simulink model "Reformable_AI_2025"  (R2025b)
settings: Solver=ode23t  StartTime=0.0  StopTime=150  FixedStep=0.01  RelTol=1e-3
InitFcn:
  | load('PV_Params_Stage1.mat'); load('PV_Params_Stage2.mat');
values from neighbouring files (symbols this model uses):
  Iph_ref = P.Iph_ref*(1 - K.k_Iph*D)    [PaperFigures.m]
  n = lower(name)    [Stage10C_inventory.m]    (also in Stage10F2_make_manifest.m = size(rows,1); Stage10F_make_manifest.m = size(rows,1); Stage10F_run_one.m = 1; Stage10_assemble_dataset.m = height(T))
  OCV_tbl = [11.6 11.8 11.9 12.1 12.2 12.3 12.4 12.5 12.6 12.7 12.8]    [Battery_Param_Definition.m]
  Q = 7    [Battery_Param_Definition.m]
  q = 1.602176634e-19    [PaperFigures.m]    (also in Stage10C_inventory.m = L(strcmp({L.folder}, fl{k})); Stage10F2_make_manifest.m = M(M.regime == "A" & abs(M.bD - L) < 1e-12, :); Stage10F_make_manifest.m = M(M.regime == "A" & abs(M.bD - L) < 1e-12, :); Stage10G2_final_test.m = zeros(1, numel(seeds)))
  R0 = 0.03    [Battery_Param_Definition.m]    (also in PaperFigures.m = B.R0*(1 + KB.k_R0*D))
  R1 = 0.015    [Battery_Param_Definition.m]    (also in PaperFigures.m = B.R1*(1 + KB.k_R1*D))
  Rs = P.Rs*(1 + K.k_Rs*D)    [PaperFigures.m]
  Rsh = P.Rsh*(1 - K.k_Rsh*D)    [PaperFigures.m]
  SOC_bp = [0 10 20 30 40 50 60 70 80 90 100]    [Battery_Param_Definition.m]
  SOC_init = 100    [Battery_Param_Definition.m]
undefined symbols (not defined in the file or in its folder): Battery_Twin_C1, Battery_Twin_Capacity, Battery_Twin_OCV_tbl, Battery_Twin_R0, Battery_Twin_R1, Battery_Twin_SOC_bp, Battery_Twin_SOC_init, Battery_Twin_Vp_init, bias_G, bias_I_batt, bias_I_pv, bias_T_batt, bias_Tc, bias_V_batt, bias_V_pv, dG, dI_batt, dI_pv, drift_G, drift_I_batt, drift_I_pv, drift_T_batt, drift_Tc, drift_V_batt, drift_V_pv, dT_batt, dTc, dV_batt, dV_pv, Eg, ExcessiveNoise_Sigma, ExcessiveNoise_Sigma_batt, ExtraDrift_Rate, ExtraDrift_Rate_batt, FaultBias_Value, FaultBias_Value_batt, FaultSat_Max, FaultSat_Max_batt, FaultSat_Min, FaultSat_Min_batt, G_max, G_min, Gref, I0_ref, I_batt_max, I_batt_min, I_pv_max, I_pv_min, IntermittentDropoutProb, IntermittentDropoutProb_batt, Isc_ref, k_B, k_Iph, k_Q, k_R0, k_R1, k_Rs, k_Rsh, Ki, noise_G ... (+44)
libraries: fl_lib x7, nesl_utility x6
(part 2 of 3)

== system Reformable_AI_2025/PV_Resdual_Model ==
  PV_Twin_Current : Inport
  PV_Twin_Power : Inport  Port=2
  PV_Measured_Power : Inport  Port=3
  PV_Measured_Current : Inport  Port=4
  MATLAB Function : MATLAB Function  TreatAsAtomicUnit=on
  To Workspace : ToWorkspace  VariableName=PV_Residual_Current  SaveFormat=Timeseries  SampleTime=-1
  To Workspace1 : ToWorkspace  VariableName=PV_Residual_Power  SaveFormat=Timeseries  SampleTime=-1
  PV_Residual_Current : Outport
  PV_Residual_Power : Outport  Port=2
  wires:
  PV_Twin_Power/1 -> MATLAB Function/4(PV_Twin_Power)
  PV_Measured_Power/1 -> MATLAB Function/3(PV_Measured_Power)
  PV_Twin_Current/1 -> MATLAB Function/2(PV_Twin_Current)
  PV_Measured_Current/1 -> MATLAB Function/1(PV_Measured_Current)
  MATLAB Function/1(PV_Residual_Current) -> To Workspace/1, PV_Residual_Current/1
  MATLAB Function/2(PV_Residual_Power) -> To Workspace1/1, PV_Residual_Power/1

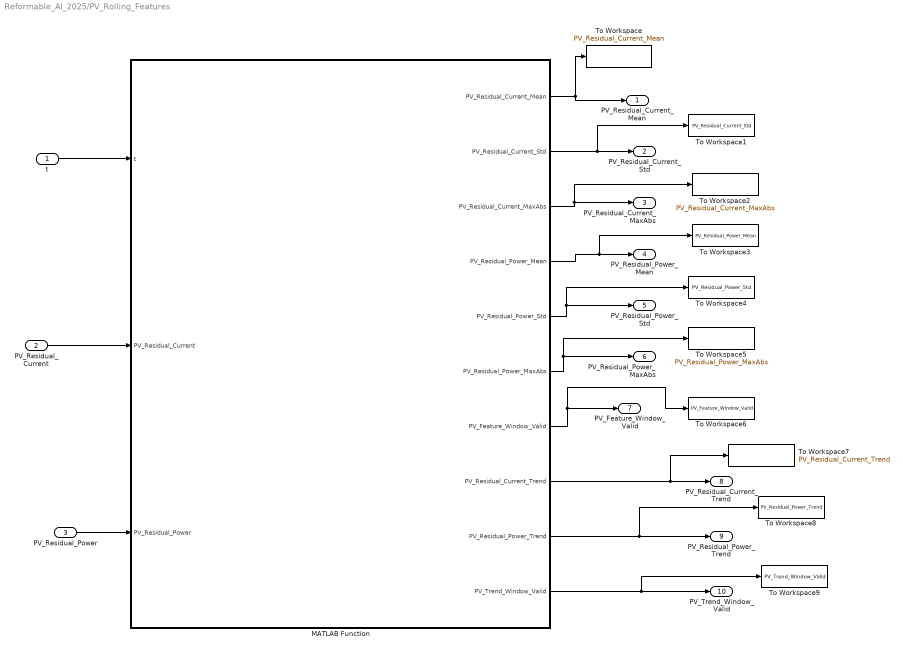
== system Reformable_AI_2025/PV_Rolling_Features ==
  t : Inport
  PV_Residual_Current : Inport  Port=2
  PV_Residual_Power : Inport  Port=3
  MATLAB Function : MATLAB Function  TreatAsAtomicUnit=on  SystemSampleTime=Stage9_Feature_SampleTime
  To Workspace : ToWorkspace  VariableName=PV_Residual_Current_Mean  SaveFormat=Timeseries  SampleTime=-1
  To Workspace1 : ToWorkspace  VariableName=PV_Residual_Current_Std  SaveFormat=Timeseries  SampleTime=-1
  To Workspace2 : ToWorkspace  VariableName=PV_Residual_Current_MaxAbs  SaveFormat=Timeseries  SampleTime=-1
  To Workspace3 : ToWorkspace  VariableName=PV_Residual_Power_Mean  SaveFormat=Timeseries  SampleTime=-1
  To Workspace4 : ToWorkspace  VariableName=PV_Residual_Power_Std  SaveFormat=Timeseries  SampleTime=-1
  To Workspace5 : ToWorkspace  VariableName=PV_Residual_Power_MaxAbs  SaveFormat=Timeseries  SampleTime=-1
  To Workspace6 : ToWorkspace  VariableName=PV_Feature_Window_Valid  SaveFormat=Timeseries  SampleTime=-1
  To Workspace7 : ToWorkspace  VariableName=PV_Residual_Current_Trend  SaveFormat=Timeseries  SampleTime=-1
  To Workspace8 : ToWorkspace  VariableName=PV_Residual_Power_Trend  SaveFormat=Timeseries  SampleTime=-1
  To Workspace9 : ToWorkspace  VariableName=PV_Trend_Window_Valid  SaveFormat=Timeseries  SampleTime=-1
  PV_Residual_Current_Mean : Outport
  PV_Residual_Current_Std : Outport  Port=2
  PV_Residual_Current_MaxAbs : Outport  Port=3
  PV_Residual_Power_Mean : Outport  Port=4
  PV_Residual_Power_Std : Outport  Port=5
  PV_Residual_Power_MaxAbs : Outport  Port=6
  PV_Feature_Window_Valid : Outport  Port=7
  PV_Residual_Current_Trend : Outport  Port=8
  PV_Residual_Power_Trend : Outport  Port=9
  PV_Trend_Window_Valid : Outport  Port=10
  wires:
  t/1 -> MATLAB Function/1(t)
  PV_Residual_Current/1 -> MATLAB Function/2(PV_Residual_Current)
  PV_Residual_Power/1 -> MATLAB Function/3(PV_Residual_Power)
  MATLAB Function/1(PV_Residual_Current_Mean) -> To Workspace/1, PV_Residual_Current_Mean/1
  MATLAB Function/2(PV_Residual_Current_Std) -> To Workspace1/1, PV_Residual_Current_Std/1
  MATLAB Function/3(PV_Residual_Current_MaxAbs) -> To Workspace2/1, PV_Residual_Current_MaxAbs/1
  MATLAB Function/4(PV_Residual_Power_Mean) -> To Workspace3/1, PV_Residual_Power_Mean/1
  MATLAB Function/5(PV_Residual_Power_Std) -> To Workspace4/1, PV_Residual_Power_Std/1
  MATLAB Function/6(PV_Residual_Power_MaxAbs) -> To Workspace5/1, PV_Residual_Power_MaxAbs/1
  MATLAB Function/7(PV_Feature_Window_Valid) -> To Workspace6/1, PV_Feature_Window_Valid/1
  MATLAB Function/8(PV_Residual_Current_Trend) -> To Workspace7/1, PV_Residual_Current_Trend/1
  MATLAB Function/9(PV_Residual_Power_Trend) -> To Workspace8/1, PV_Residual_Power_Trend/1
  MATLAB Function/10(PV_Trend_Window_Valid) -> To Workspace9/1, PV_Trend_Window_Valid/1

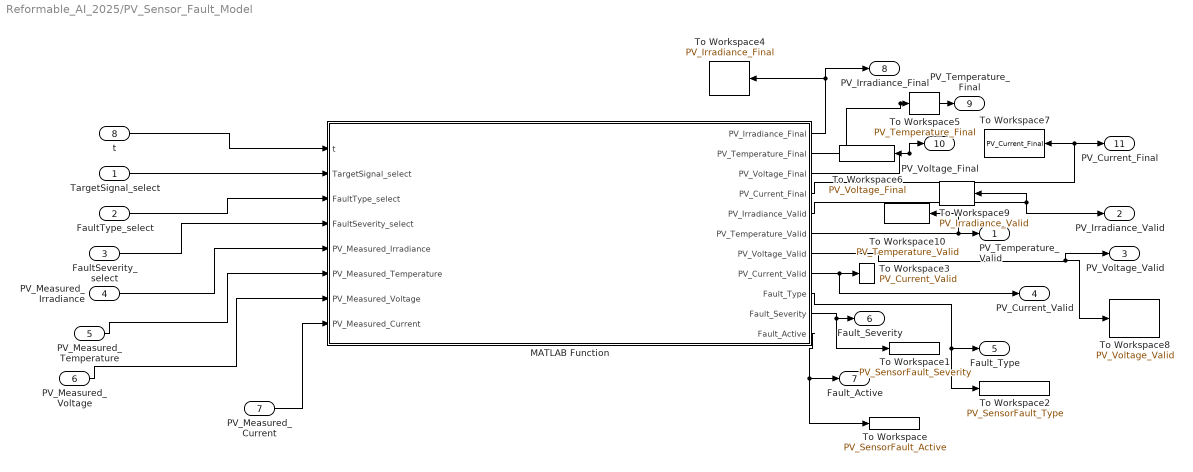
== system Reformable_AI_2025/PV_Sensor_Fault_Model ==
  TargetSignal_select : Inport
  FaultType_select : Inport  Port=2
  FaultSeverity_select : Inport  Port=3
  PV_Measured_Irradiance : Inport  Port=4
  PV_Measured_Temperature : Inport  Port=5
  PV_Measured_Voltage : Inport  Port=6
  PV_Measured_Current : Inport  Port=7
  t : Inport  Port=8
  MATLAB Function : MATLAB Function  TreatAsAtomicUnit=on
  To Workspace : ToWorkspace  VariableName=PV_SensorFault_Active  SaveFormat=Timeseries  SampleTime=-1
  To Workspace1 : ToWorkspace  VariableName=PV_SensorFault_Severity  SaveFormat=Timeseries  SampleTime=-1
  To Workspace10 : ToWorkspace  VariableName=PV_Temperature_Valid  SaveFormat=Timeseries  SampleTime=-1
  To Workspace2 : ToWorkspace  VariableName=PV_SensorFault_Type  SaveFormat=Timeseries  SampleTime=-1
  To Workspace3 : ToWorkspace  VariableName=PV_Current_Valid  SaveFormat=Timeseries  SampleTime=-1
  To Workspace4 : ToWorkspace  VariableName=PV_Irradiance_Final  SaveFormat=Timeseries  SampleTime=-1
  To Workspace5 : ToWorkspace  VariableName=PV_Temperature_Final  SaveFormat=Timeseries  SampleTime=-1
  To Workspace6 : ToWorkspace  VariableName=PV_Voltage_Final  SaveFormat=Timeseries  SampleTime=-1
  To Workspace7 : ToWorkspace  VariableName=PV_Current_Final  SaveFormat=Timeseries  SampleTime=-1
  To Workspace8 : ToWorkspace  VariableName=PV_Voltage_Valid  SaveFormat=Timeseries  SampleTime=-1
  To Workspace9 : ToWorkspace  VariableName=PV_Irradiance_Valid  SaveFormat=Timeseries  SampleTime=-1
  PV_Temperature_Valid : Outport
  PV_Irradiance_Valid : Outport  Port=2
  PV_Voltage_Valid : Outport  Port=3
  PV_Current_Valid : Outport  Port=4
  Fault_Type : Outport  Port=5
  Fault_Severity : Outport  Port=6
  Fault_Active : Outport  Port=7
  PV_Irradiance_Final : Outport  Port=8
  PV_Temperature_Final : Outport  Port=9
  PV_Voltage_Final : Outport  Port=10
  PV_Current_Final : Outport  Port=11
  wires:
  t/1 -> MATLAB Function/1(t)
  TargetSignal_select/1 -> MATLAB Function/2(TargetSignal_select)
  FaultType_select/1 -> MATLAB Function/3(FaultType_select)
  FaultSeverity_select/1 -> MATLAB Function/4(FaultSeverity_select)
  PV_Measured_Irradiance/1 -> MATLAB Function/5(PV_Measured_Irradiance)
  PV_Measured_Temperature/1 -> MATLAB Function/6(PV_Measured_Temperature)
  PV_Measured_Voltage/1 -> MATLAB Function/7(PV_Measured_Voltage)
  PV_Measured_Current/1 -> MATLAB Function/8(PV_Measured_Current)
  MATLAB Function/1(PV_Irradiance_Final) -> To Workspace4/1, PV_Irradiance_Final/1
  MATLAB Function/2(PV_Temperature_Final) -> To Workspace5/1, PV_Temperature_Final/1
  MATLAB Function/3(PV_Voltage_Final) -> PV_Voltage_Final/1, To Workspace6/1
  MATLAB Function/4(PV_Current_Final) -> PV_Current_Final/1, To Workspace7/1
  MATLAB Function/5(PV_Irradiance_Valid) -> PV_Irradiance_Valid/1, To Workspace9/1
  MATLAB Function/6(PV_Temperature_Valid) -> To Workspace10/1, PV_Temperature_Valid/1
  MATLAB Function/7(PV_Voltage_Valid) -> To Workspace8/1, PV_Voltage_Valid/1
  MATLAB Function/8(PV_Current_Valid) -> PV_Current_Valid/1, To Workspace3/1
  MATLAB Function/9(Fault_Type) -> Fault_Type/1, To Workspace2/1
  MATLAB Function/10(Fault_Severity) -> To Workspace1/1, Fault_Severity/1
  MATLAB Function/11(Fault_Active) -> Fault_Active/1, To Workspace/1

== system Reformable_AI_2025/PV_Twin_Valid_Operating_Point ==
  PV_Measured_Voltage : Inport
  PV_Measured_Irradiance : Inport  Port=2
  PV_Twin_Current : Inport  Port=3
  PV_Twin_Power : Inport  Port=4
  MATLAB Function : MATLAB Function  TreatAsAtomicUnit=on
  To Workspace : ToWorkspace  VariableName=PV_Twin_Valid_Operating_Point  SaveFormat=Timeseries  SampleTime=-1
  PV_Twin_Valid_Operating_Point : Outport
  wires:
  MATLAB Function/1(PV_Twin_Valid_Operating_Point) -> To Workspace/1, PV_Twin_Valid_Operating_Point/1
  PV_Measured_Voltage/1 -> MATLAB Function/1(PV_Measured_Voltage)
  PV_Measured_Irradiance/1 -> MATLAB Function/2(PV_Measured_Irradiance)
  PV_Twin_Current/1 -> MATLAB Function/3(PV_Twin_Current)
  PV_Twin_Power/1 -> MATLAB Function/4(PV_Twin_Power)

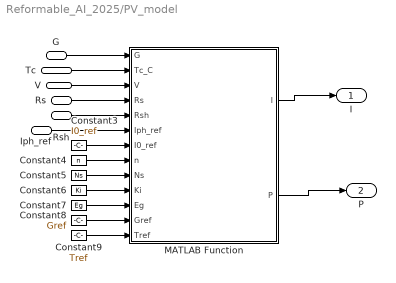
== system Reformable_AI_2025/PV_model ==
  G : Inport
  Tc : Inport  Port=2
  V : Inport  Port=3
  Rs : Inport  Port=4
  Rsh : Inport  Port=5
  Iph_ref : Inport  Port=6
  Constant3 : Constant  Value=I0_ref
  Constant4 : Constant  Value=n
  Constant5 : Constant  Value=Ns
  Constant6 : Constant  Value=Ki
  Constant7 : Constant  Value=Eg
  Constant8 : Constant  Value=Gref
  Constant9 : Constant  Value=Tref
  MATLAB Function : MATLAB Function  TreatAsAtomicUnit=on
  I : Outport
  P : Outport  Port=2
  wires:
  MATLAB Function/1(I) -> I/1
  G/1 -> MATLAB Function/1(G)
  Tc/1 -> MATLAB Function/2(Tc_C)
  V/1 -> MATLAB Function/3(V)
  MATLAB Function/2(P) -> P/1
  Rs/1 -> MATLAB Function/4(Rs)
  Rsh/1 -> MATLAB Function/5(Rsh)
  Iph_ref/1 -> MATLAB Function/6(Iph_ref)
  Constant3/1 -> MATLAB Function/7(I0_ref)
  Constant4/1 -> MATLAB Function/8(n)
  Constant5/1 -> MATLAB Function/9(Ns)
  Constant6/1 -> MATLAB Function/10(Ki)
  Constant7/1 -> MATLAB Function/11(Eg)
  Constant9/1 -> MATLAB Function/13(Tref)
  Constant8/1 -> MATLAB Function/12(Gref)

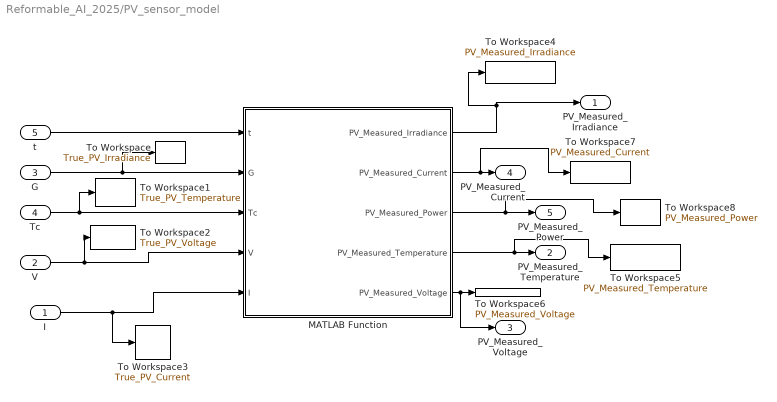
== system Reformable_AI_2025/PV_sensor_model ==
  I : Inport
  V : Inport  Port=2
  G : Inport  Port=3
  Tc : Inport  Port=4
  t : Inport  Port=5
  MATLAB Function : MATLAB Function  TreatAsAtomicUnit=on
  To Workspace : ToWorkspace  VariableName=True_PV_Irradiance  SaveFormat=Timeseries  SampleTime=-1
  To Workspace1 : ToWorkspace  VariableName=True_PV_Temperature  SaveFormat=Timeseries  SampleTime=-1
  To Workspace2 : ToWorkspace  VariableName=True_PV_Voltage  SaveFormat=Timeseries  SampleTime=-1
  To Workspace3 : ToWorkspace  VariableName=True_PV_Current  SaveFormat=Timeseries  SampleTime=-1
  To Workspace4 : ToWorkspace  VariableName=PV_Measured_Irradiance  SaveFormat=Timeseries  SampleTime=-1
  To Workspace5 : ToWorkspace  VariableName=PV_Measured_Temperature  SaveFormat=Timeseries  SampleTime=-1
  To Workspace6 : ToWorkspace  VariableName=PV_Measured_Voltage  SaveFormat=Timeseries  SampleTime=-1
  To Workspace7 : ToWorkspace  VariableName=PV_Measured_Current  SaveFormat=Timeseries  SampleTime=-1
  To Workspace8 : ToWorkspace  VariableName=PV_Measured_Power  SaveFormat=Timeseries  SampleTime=-1
  PV_Measured_Irradiance : Outport
  PV_Measured_Temperature : Outport  Port=2
  PV_Measured_Voltage : Outport  Port=3
  PV_Measured_Current : Outport  Port=4
  PV_Measured_Power : Outport  Port=5
  wires:
  Tc/1 -> To Workspace1/1, MATLAB Function/3(Tc)
  G/1 -> To Workspace/1, MATLAB Function/2(G)
  V/1 -> To Workspace2/1, MATLAB Function/4(V)
  t/1 -> MATLAB Function/1(t)
  MATLAB Function/1(PV_Measured_Irradiance) -> To Workspace4/1, PV_Measured_Irradiance/1
  I/1 -> To Workspace3/1, MATLAB Function/5(I)
  MATLAB Function/5(PV_Measured_Voltage) -> PV_Measured_Voltage/1, To Workspace6/1
  MATLAB Function/2(PV_Measured_Current) -> To Workspace7/1, PV_Measured_Current/1
  MATLAB Function/3(PV_Measured_Power) -> To Workspace8/1, PV_Measured_Power/1
  MATLAB Function/4(PV_Measured_Temperature) -> To Workspace5/1, PV_Measured_Temperature/1

== matlab function Reformable_AI_2025/PV_Fault_Model/MATLAB Function ==
  data: t input; Rs_fault output; Rs_aged input; Rsh_aged input; Iph_ref_aged input; FaultType_select input; FaultSeverity_select input; Rsh_fault output; Iph_fault output; Fault_Type output; Fault_Severity output; Fault_Active output; Fault_TempRise output
function [Rs_fault, Rsh_fault, Iph_fault, Fault_Type, Fault_Severity, Fault_Active, Fault_TempRise] = ...
    fcn(t, Rs_aged, Rsh_aged, Iph_ref_aged, FaultType_select, FaultSeverity_select)

% TwinAdapt-PHM Stage 5: PV Fault Injection
% Faults modify DEGRADED (aged) parameters, never nameplate/reference values.
% FaultType_select: 0=Healthy 1=Shading 2=Soiling 3=Hotspot 4=PID 5=OpenCircuit 6=ShortCircuit
% FaultSeverity_select: 0 (no fault) to 1 (fully severe)

s = max(0, min(1, FaultSeverity_select));  % clamp severity to [0,1]
ft = round(FaultType_select);

% Defaults: pass-through (Healthy)
Rs_fault  = Rs_aged;
Rsh_fault = Rsh_aged;
Iph_fault = Iph_ref_aged;
Fault_TempRise = 0;
Fault_Active = (ft ~= 0) && (s > 0);

switch ft

    case 0  % Healthy
        Fault_Type = 0;
        Fault_Severity = 0;

    case 1  % Partial Shading -> reduces Iph
        ShadeFactor = s;                      % up to 100% reduction at s=1
        Iph_fault = Iph_ref_aged * (1 - ShadeFactor);
        Fault_Type = 1;
        Fault_Severity = s;

    case 2  % Soiling -> mild Iph reduction + slight temp rise
        Iph_fault = Iph_ref_aged * (1 - 0.3*s);   % gentler than shading
        Fault_TempRise = 5 * s;                   % degC, gradual heating
        Fault_Type = 2;
        Fault_Severity = s;

    case 3  % Hotspot -> increases Rs, raises temperature
        k_hotspot = 4.0;                          % tunable multiplier gain
        Rs_fault = Rs_aged * (1 + k_hotspot*s);
        Fault_TempRise = 40 * s;                   % degC, hotspots run hot
        Fault_Type = 3;
        Fault_Severity = s;

    case 4  % PID -> collapses Rsh (leakage current path)
        k_pid = 0.95;                              % up to 95% Rsh reduction
        Rsh_fault = Rsh_aged * (1 - k_pid*s);
        Fault_Type = 4;
        Fault_Severity = s;

    case 5  % Open Circuit -> current forced to ~0
        Iph_fault = Iph_ref_aged * (1 - s);         % s=1 -> Iph~0 -> I~0, V~Voc
        Rs_fault = Rs_aged * (1 + 50*s);            % huge series resistance emulates open ckt
        Fault_Type = 5;
        Fault_Severity = s;

    case 6  % Short Circuit -> voltage forced to ~0
        Rsh_fault = Rsh_aged * (1 - 0.999*s);       % Rsh -> ~0 collapses voltage
        Fault_Type = 6;
        Fault_Severity = s;

    otherwise  % unrecognized code -> treat as Healthy, flag inactive
        Fault_Type = 0;
        Fault_Severity = 0;
        Fault_Active = false;
end

end

== matlab function Reformable_AI_2025/Battery_Fault_Model/MATLAB Function ==
  data: t input; R0_fault output; R0_aged input; R1_aged input; Q input; OCV_delta input; D_batt input; H_batt input; Battery_Health_State input; FaultType_select input; FaultSeverity_select input; R1_fault output; Q_fault output; OCV_delta_fault output; D_batt output; H_batt output; Battery_Health_State output; Fault_Type output; Fault_Severity output; Fault_Active output; Battery_TempRise output; Safety_Flag output; SafetyFlag_Warning_ThresholdC parameter; SafetyFlag_Critical_ThresholdC parameter; SafetyFlag_Emergency_ThresholdC parameter; k_open_R0 parameter; TempRise_short parameter; k_short_R0 parameter; TempRise_runaway parameter; k_runaway_R0 parameter; TempRise_overcharge parameter; k_overcharge_OCV parameter; k_overcharge_R1 parameter; k_overdischarge_R0 parameter; k_overdischarge_Q parameter; TempRise_overdischarge parameter; TempRise_imbalance parameter; k_imbalance_OCV parameter; k_imbalance_R0 parameter
function [R0_fault, R1_fault, Q_fault, OCV_delta_fault, D_batt, H_batt, ...
          Battery_Health_State, Fault_Type, Fault_Severity, Fault_Active, ...
          Battery_TempRise, Safety_Flag] = ...
    fcn(t, R0_aged, R1_aged, Q, OCV_delta, D_batt, H_batt, ...
          Battery_Health_State, FaultType_select, FaultSeverity_select, ...
        SafetyFlag_Warning_ThresholdC, SafetyFlag_Critical_ThresholdC, SafetyFlag_Emergency_ThresholdC, k_open_R0, ...
TempRise_short, ...
k_short_R0, TempRise_runaway, ...
k_runaway_R0, TempRise_overcharge, ...
k_overcharge_OCV, k_overcharge_R1, k_overdischarge_R0, k_overdischarge_Q, TempRise_overdischarge, ...
TempRise_imbalance, ...
k_imbalance_OCV, k_imbalance_R0)

% TwinAdapt-PHM Stage 6: Battery Fault Injection
% Faults modify DEGRADED (aged) parameters, never nameplate/reference values.
% FaultType_select: 0=Healthy 1=CellImbalance 2=OverDischarge 3=OverCharge
%                   4=ThermalRunawayOnset 5=InternalShort 6=OpenCircuit
%                   7=SensorFault (placeholder -- see note below)
%
% NOTE ON SYMBOLS PANE: everything after FaultSeverity_select in the
% argument list above must have its Scope set to "Parameter" in the
% Ports and Data Manager, NOT "Input". Only the first 10 arguments
% (t through FaultSeverity_select) should be Scope = Input.

s = max(0, min(1, FaultSeverity_select));  % clamp severity to [0,1]
ft = round(FaultType_select);

% Defaults: pass-through (Healthy)
R0_fault         = R0_aged;
R1_fault         = R1_aged;
Q_fault          = Q;
OCV_delta_fault  = OCV_delta;
Battery_TempRise = 0;
Fault_Active     = (ft ~= 0) && (s > 0);

switch ft

    case 0  % Healthy
        Fault_Type = 0;
        Fault_Severity = 0;

    case 1  % Cell Imbalance -> mild R0 rise, OCV uncertainty band
        R0_fault = R0_aged * (1 + k_imbalance_R0*s);
        OCV_delta_fault = OCV_delta + k_imbalance_OCV*s;
        Battery_TempRise = TempRise_imbalance * s;
        Fault_Type = 1;
        Fault_Severity = s;

    case 2  % Over-Discharge -> permanent capacity loss, R0 rise
        Q_fault = Q * (1 - k_overdischarge_Q*s);
        R0_fault = R0_aged * (1 + k_overdischarge_R0*s);
        Battery_TempRise = TempRise_overdischarge * s;
        Fault_Type = 2;
        Fault_Severity = s;

    case 3  % Over-Charge -> R1 rise, small OCV increase, heating
        R1_fault = R1_aged * (1 + k_overcharge_R1*s);
        OCV_delta_fault = OCV_delta + k_overcharge_OCV*s;
        Battery_TempRise = TempRise_overcharge * s;
        Fault_Type = 3;
        Fault_Severity = s;

    case 4  % Thermal Runaway Onset -> rapid R0 rise, severe heating
        R0_fault = R0_aged * (1 + k_runaway_R0*s);
        Battery_TempRise = TempRise_runaway * s;
        Fault_Type = 4;
        Fault_Severity = s;

    case 5  % Internal Short -> R0 collapses toward zero, current spikes
        R0_fault = R0_aged * (1 - k_short_R0*s);
        Battery_TempRise = TempRise_short * s;
        Fault_Type = 5;
        Fault_Severity = s;

    case 6  % Open Circuit -> R0 inflated to emulate disconnection
        R0_fault = R0_aged * (1 + k_open_R0*s);
        Battery_TempRise = 0;
        Fault_Type = 6;
        Fault_Severity = s;

    case 7  % Sensor Fault -- PLACEHOLDER ONLY
        % Physics intentionally untouched. This fault type is architecturally
        % downstream of Battery_Model (biases Terminal_voltage/Battery_Current/
        % T_batt readings, which don't exist yet at this point in the pipeline).
        % Recognized here so FaultType_select=7 doesn't fall through to
        % 'otherwise', but real sensor-bias logic belongs in a future
        % Battery_Sensor_Fault_Model placed after Battery_Model.
        Fault_Type = 7;
        Fault_Severity = s;

    otherwise  % unrecognized code -> treat as Healthy, flag inactive
        Fault_Type = 0;
        Fault_Severity = 0;
        Fault_Active = false;
end

% Safety_Flag: derived from Battery_TempRise, thresholds tuned to this
% library's actual max TempRise (40 degC at Thermal Runaway, s=1)
if Battery_TempRise > SafetyFlag_Emergency_ThresholdC
    Safety_Flag = 3;
elseif Battery_TempRise > SafetyFlag_Critical_ThresholdC
    Safety_Flag = 2;
elseif Battery_TempRise > SafetyFlag_Warning_ThresholdC
    Safety_Flag = 1;
else
    Safety_Flag = 0;
end

end

== matlab function Reformable_AI_2025/PV_sensor_model/MATLAB Function ==
  settings: updateMethod=DISCRETE
  data: t input; PV_Measured_Irradiance output; PV_Measured_Current output; PV_Measured_Power output; PV_Measured_Temperature output; PV_Measured_Voltage output; G input; Tc input; V input; I input; noise_G parameter; bias_G parameter; drift_G parameter; dG parameter; G_min parameter; G_max parameter; noise_Tc parameter; bias_Tc parameter; drift_Tc parameter; dTc parameter; Tc_min parameter; Tc_max parameter; noise_V_pv parameter; bias_V_pv parameter; drift_V_pv parameter; dV_pv parameter; V_pv_min parameter; V_pv_max parameter; noise_I_pv parameter; bias_I_pv parameter; drift_I_pv parameter; dI_pv parameter; I_pv_min parameter; I_pv_max parameter
function [PV_Measured_Irradiance, PV_Measured_Current, PV_Measured_Power, PV_Measured_Temperature, PV_Measured_Voltage] ...
= ...
    fcn(t, G, Tc, V, I, ...
        noise_G, bias_G, drift_G, dG, G_min, G_max, ...
noise_Tc, bias_Tc, drift_Tc, dTc, Tc_min, Tc_max, ...
noise_V_pv, bias_V_pv, drift_V_pv, dV_pv, V_pv_min, V_pv_max, ...
noise_I_pv, bias_I_pv, drift_I_pv, dI_pv, I_pv_min, I_pv_max)

% TwinAdapt-PHM Stage 7 (Step 1): PV_Sensor_Model
% Baseline sensor realism ONLY -- no fault injection here (that's a later
% step, PV_Sensor_Fault_Model). Signal chain per quantity:
%   True value -> + bias(t) [bias + drift*t] -> + Gaussian noise
%               -> saturate to sensor range -> quantize to ADC resolution
%
% NOTE ON SYMBOLS PANE: t, G, Tc, V, I must be Scope = Input.
% Every argument after I (all noise/bias/drift/dX/min/max terms) must be
% Scope = Parameter, resolved from the base workspace (PV_Sensor_Params.mat).
%
% PV_Measured_Power is intentionally NOT independently noised/quantized --
% it's derived from the already-processed Measured_Voltage and
% Measured_Current, matching how a real deployed system computes power
% from its actual V/I sensors rather than having a dedicated power sensor.

% --- Irradiance ---
G_biased = G + bias_G + drift_G*t;
G_noisy  = G_biased + noise_G*randn;
G_sat    = min(max(G_noisy, G_min), G_max);
PV_Measured_Irradiance = round(G_sat/dG)*dG;

% --- Module temperature ---
Tc_biased = Tc + bias_Tc + drift_Tc*t;
Tc_noisy  = Tc_biased + noise_Tc*randn;
Tc_sat    = min(max(Tc_noisy, Tc_min), Tc_max);
PV_Measured_Temperature = round(Tc_sat/dTc)*dTc;

% --- PV voltage ---
V_biased = V + bias_V_pv + drift_V_pv*t;
V_noisy  = V_biased + noise_V_pv*randn;
V_sat    = min(max(V_noisy, V_pv_min), V_pv_max);
PV_Measured_Voltage = round(V_sat/dV_pv)*dV_pv;

% --- PV current ---
I_biased = I + bias_I_pv + drift_I_pv*t;
I_noisy  = I_biased + noise_I_pv*randn;
I_sat    = min(max(I_noisy, I_pv_min), I_pv_max);
PV_Measured_Current = round(I_sat/dI_pv)*dI_pv;

% --- PV power, derived (not independently sensed) ---
PV_Measured_Power = PV_Measured_Voltage * PV_Measured_Current;

end

== matlab function Reformable_AI_2025/PV_Sensor_Fault_Model/MATLAB Function ==
  settings: updateMethod=DISCRETE
  data: t input; TargetSignal_select input; PV_Irradiance_Final output; FaultType_select input; FaultSeverity_select input; PV_Measured_Irradiance input; PV_Measured_Temperature input; PV_Measured_Voltage input; PV_Measured_Current input; PV_Temperature_Final output; PV_Voltage_Final output; PV_Current_Final output; PV_Irradiance_Valid output; PV_Temperature_Valid output; PV_Voltage_Valid output; PV_Current_Valid output; Fault_Type output; Fault_Severity output; Fault_Active output; StuckAt_G parameter; StuckAt_Tc parameter; StuckAt_V_pv parameter; StuckAt_I_pv parameter; IntermittentDropoutProb parameter; FaultSat_Min parameter; FaultSat_Max parameter; ExcessiveNoise_Sigma parameter; ExtraDrift_Rate parameter; FaultBias_Value parameter
function [PV_Irradiance_Final, PV_Temperature_Final, PV_Voltage_Final, PV_Current_Final, ...
          PV_Irradiance_Valid, PV_Temperature_Valid, PV_Voltage_Valid, PV_Current_Valid, ...
          Fault_Type, Fault_Severity, Fault_Active] = ...
    fcn(t, TargetSignal_select, FaultType_select, FaultSeverity_select, ...
        PV_Measured_Irradiance, PV_Measured_Temperature, PV_Measured_Voltage, PV_Measured_Current, ...
        StuckAt_G, StuckAt_Tc, StuckAt_V_pv, StuckAt_I_pv, ...
        IntermittentDropoutProb, FaultSat_Min, FaultSat_Max, ...
        ExcessiveNoise_Sigma, ExtraDrift_Rate, FaultBias_Value)

% TwinAdapt-PHM Stage 7 (Step 2): PV_Sensor_Fault_Model
% Measurement-layer faults ONLY -- sits after PV_Sensor_Model. Does NOT
% touch physical asset health (that's PV_Fault_Model, Stage 5). Applies
% ONE selected fault to ONE selected target channel per run; the other
% three channels pass through unchanged.
%
% FaultType_select:    0=Healthy 1=Bias(extra) 2=StuckAt 3=Dropout
%                      4=Intermittent 5=ForcedSaturation 6=ExcessiveNoise
%                      7=ExtraDrift
% TargetSignal_select: 0=Irradiance 1=Temperature 2=Voltage 3=Current
%
% NOTE ON SYMBOLS PANE: t, TargetSignal_select, FaultType_select,
% FaultSeverity_select, PV_Measured_Irradiance, PV_Measured_Temperature,
% PV_Measured_Voltage, PV_Measured_Current must be Scope = Input.
% Everything after that (StuckAt_G ... FaultBias_Value) must be
% Scope = Parameter, resolved from PV_Sensor_Fault_Params.mat.

% Defaults: pass-through, everything valid
PV_Irradiance_Final  = PV_Measured_Irradiance;
PV_Temperature_Final = PV_Measured_Temperature;
PV_Voltage_Final     = PV_Measured_Voltage;
PV_Current_Final     = PV_Measured_Current;
PV_Irradiance_Valid  = true;
PV_Temperature_Valid = true;
PV_Voltage_Valid     = true;
PV_Current_Valid     = true;

s      = max(0, min(1, FaultSeverity_select));
ft     = round(FaultType_select);
target = round(TargetSignal_select);

Fault_Type     = ft;
Fault_Severity = s;
Fault_Active   = (ft ~= 0) && (s > 0);

if Fault_Active
    % Select which channel's true value and stuck-at constant apply
    switch target
        case 0
            trueVal  = PV_Measured_Irradiance;
            stuckVal = StuckAt_G;
        case 1
            trueVal  = PV_Measured_Temperature;
            stuckVal = StuckAt_Tc;
        case 2
            trueVal  = PV_Measured_Voltage;
            stuckVal = StuckAt_V_pv;
        case 3
            trueVal  = PV_Measured_Current;
            stuckVal = StuckAt_I_pv;
        otherwise
            trueVal  = 0;
            stuckVal = 0;
    end

    valid = true;
    switch ft
        case 1  % Bias -- extra fixed offset on top of baseline sensor bias
            faultedVal = trueVal + FaultBias_Value*s;
        case 2  % Stuck-At -- sensor frozen at a fixed reading
            faultedVal = stuckVal;
        case 3  % Dropout -- measurement lost entirely
            faultedVal = NaN;
            valid = false;
        case 4  % Intermittent -- randomly drops per-sample, probability scales with severity
            if rand < IntermittentDropoutProb*s
                faultedVal = NaN;
                valid = false;
            else
                faultedVal = trueVal;
            end
        case 5  % Forced Saturation -- clip to an abnormal (test-configured) range
            faultedVal = min(max(trueVal, FaultSat_Min), FaultSat_Max);
        case 6  % Excessive Noise -- large extra noise beyond baseline sensor noise
            faultedVal = trueVal + ExcessiveNoise_Sigma*s*randn;
        case 7  % Extra Drift -- fast-growing bias beyond baseline sensor drift
            faultedVal = trueVal + ExtraDrift_Rate*s*t;
        otherwise
            faultedVal = trueVal;
    end

    % Write the faulted value/valid-flag back into only the targeted channel
    switch target
        case 0
            PV_Irradiance_Final = faultedVal;
            PV_Irradiance_Valid = valid;
        case 1
            PV_Temperature_Final = faultedVal;
            PV_Temperature_Valid = valid;
        case 2
            PV_Voltage_Final = faultedVal;
            PV_Voltage_Valid = valid;
        case 3
            PV_Current_Final = faultedVal;
            PV_Current_Valid = valid;
    end
end

end

== matlab function Reformable_AI_2025/Battery_Sensor_Model/MATLAB Function ==
  settings: updateMethod=DISCRETE
  data: t input; Battery_Measured_Voltage output; Terminal_voltage input; Battery_Current input; T_batt input; noise_V_batt parameter; bias_V_batt parameter; drift_V_batt parameter; dV_batt parameter; V_batt_min parameter; V_batt_max parameter; noise_I_batt parameter; bias_I_batt parameter; drift_I_batt parameter; dI_batt parameter; I_batt_min parameter; I_batt_max parameter; noise_T_batt parameter; bias_T_batt parameter; drift_T_batt parameter; dT_batt parameter; T_batt_min parameter; T_batt_max parameter; Battery_Measured_Current output; Battery_Measured_Temperature output
function [Battery_Measured_Voltage, Battery_Measured_Current, Battery_Measured_Temperature] = ...
    fcn(t, Terminal_voltage, Battery_Current, T_batt, ...
        noise_V_batt, bias_V_batt, drift_V_batt, dV_batt, V_batt_min, V_batt_max, ...
        noise_I_batt, bias_I_batt, drift_I_batt, dI_batt, I_batt_min, I_batt_max, ...
        noise_T_batt, bias_T_batt, drift_T_batt, dT_batt, T_batt_min, T_batt_max)

% TwinAdapt-PHM Stage 7 (Step 3): Battery_Sensor_Model
% Baseline sensor realism ONLY -- no fault injection here (that's a later
% step, Battery_Sensor_Fault_Model). Signal chain per quantity, same as
% PV_Sensor_Model:
%   True value -> + bias(t) [bias + drift*t] -> + Gaussian noise
%               -> saturate to sensor range -> quantize to ADC resolution
%
% NOTE ON SYMBOLS PANE: t, Terminal_voltage, Battery_Current, T_batt must
% be Scope = Input. Every argument after T_batt (all noise/bias/drift/dX/
% min/max terms) must be Scope = Parameter, resolved from the base
% workspace (Battery_Sensor_Params.mat).
%
% NOTE: unlike PV, there is no derived "Battery_Measured_Power" here --
% the doc explicitly says NOT to create an artificial SOC sensor, and by
% the same reasoning we don't manufacture a battery power measurement
% this stage didn't ask for. Power/SOC estimation is a future stage's job.

% --- Battery terminal voltage ---
V_biased = Terminal_voltage + bias_V_batt + drift_V_batt*t;
V_noisy  = V_biased + noise_V_batt*randn;
V_sat    = min(max(V_noisy, V_batt_min), V_batt_max);
Battery_Measured_Voltage = round(V_sat/dV_batt)*dV_batt;

% --- Battery current ---
I_biased = Battery_Current + bias_I_batt + drift_I_batt*t;
I_noisy  = I_biased + noise_I_batt*randn;
I_sat    = min(max(I_noisy, I_batt_min), I_batt_max);
Battery_Measured_Current = round(I_sat/dI_batt)*dI_batt;

% --- Battery temperature ---
T_biased = T_batt + bias_T_batt + drift_T_batt*t;
T_noisy  = T_biased + noise_T_batt*randn;
T_sat    = min(max(T_noisy, T_batt_min), T_batt_max);
Battery_Measured_Temperature = round(T_sat/dT_batt)*dT_batt;

end

== matlab function Reformable_AI_2025/Battery_Sensor_Fault_Model/MATLAB Function ==
  settings: updateMethod=DISCRETE
  data: t input; Battery_Voltage_Final output; TargetSignal_select input; FaultType_select input; FaultSeverity_select input; Battery_Measured_Voltage input; Battery_Measured_Current input; Battery_Measured_Temperature input; Battery_Current_Final output; Battery_Temperature_Final output; Battery_Voltage_Valid output; Battery_Current_Valid output; Battery_Temperature_Valid output; Fault_Type output; Fault_Severity output; Fault_Active output; StuckAt_V_batt parameter; StuckAt_I_batt parameter; StuckAt_T_batt parameter; IntermittentDropoutProb_batt parameter; FaultSat_Min_batt parameter; FaultSat_Max_batt parameter; ExcessiveNoise_Sigma_batt parameter; ExtraDrift_Rate_batt parameter; FaultBias_Value_batt parameter
function [Battery_Voltage_Final, Battery_Current_Final, Battery_Temperature_Final, ...
          Battery_Voltage_Valid, Battery_Current_Valid, Battery_Temperature_Valid, ...
          Fault_Type, Fault_Severity, Fault_Active] = ...
    fcn(t, TargetSignal_select, FaultType_select, FaultSeverity_select, ...
        Battery_Measured_Voltage, Battery_Measured_Current, Battery_Measured_Temperature, ...
        StuckAt_V_batt, StuckAt_I_batt, StuckAt_T_batt, ...
IntermittentDropoutProb_batt, FaultSat_Min_batt, FaultSat_Max_batt, ...
ExcessiveNoise_Sigma_batt, ExtraDrift_Rate_batt, FaultBias_Value_batt)

% TwinAdapt-PHM Stage 7 (Step 4): Battery_Sensor_Fault_Model
% Measurement-layer faults ONLY -- sits after Battery_Sensor_Model. Does
% NOT touch physical asset health (that's Battery_Fault_Model, Stage 6).
% Applies ONE selected fault to ONE selected target channel per run; the
% other two channels pass through unchanged. Mirrors PV_Sensor_Fault_Model
% exactly, but with 3 channels instead of 4 (no irradiance equivalent here).
%
% FaultType_select:    0=Healthy 1=Bias(extra) 2=StuckAt 3=Dropout
%                      4=Intermittent 5=ForcedSaturation 6=ExcessiveNoise
%                      7=ExtraDrift
% TargetSignal_select: 0=Voltage 1=Current 2=Temperature
%
% NOTE ON SYMBOLS PANE: t, TargetSignal_select, FaultType_select,
% FaultSeverity_select, Battery_Measured_Voltage, Battery_Measured_Current,
% Battery_Measured_Temperature must be Scope = Input. Everything after
% that (StuckAt_V_batt ... FaultBias_Value_batt) must be Scope = Parameter,
% resolved from Battery_Sensor_Fault_Params.mat.

% Defaults: pass-through, everything valid
Battery_Voltage_Final     = Battery_Measured_Voltage;
Battery_Current_Final     = Battery_Measured_Current;
Battery_Temperature_Final = Battery_Measured_Temperature;
Battery_Voltage_Valid     = true;
Battery_Current_Valid     = true;
Battery_Temperature_Valid = true;

s      = max(0, min(1, FaultSeverity_select));
ft     = round(FaultType_select);
target = round(TargetSignal_select);

Fault_Type     = ft;
Fault_Severity = s;
Fault_Active   = (ft ~= 0) && (s > 0);

if Fault_Active
    % Select which channel's true value and stuck-at constant apply
    switch target
        case 0
            trueVal  = Battery_Measured_Voltage;
            stuckVal = StuckAt_V_batt;
        case 1
            trueVal  = Battery_Measured_Current;
            stuckVal = StuckAt_I_batt;
        case 2
            trueVal  = Battery_Measured_Temperature;
            stuckVal = StuckAt_T_batt;
        otherwise
            trueVal  = 0;
            stuckVal = 0;
    end

    valid = true;
    switch ft
        case 1  % Bias -- extra fixed offset on top of baseline sensor bias
            faultedVal = trueVal + FaultBias_Value_batt*s;
        case 2  % Stuck-At -- sensor frozen at a fixed reading
            faultedVal = stuckVal;
        case 3  % Dropout -- measurement lost entirely
            faultedVal = NaN;
            valid = false;
        case 4  % Intermittent -- randomly drops per-sample, probability scales with severity
            if rand < IntermittentDropoutProb_batt*s
                faultedVal = NaN;
                valid = false;
            else
                faultedVal = trueVal;
            end
        case 5  % Forced Saturation -- clip to an abnormal (test-configured) range
            faultedVal = min(max(trueVal, FaultSat_Min_batt), FaultSat_Max_batt);
        case 6  % Excessive Noise -- large extra noise beyond baseline sensor noise
            faultedVal = trueVal + ExcessiveNoise_Sigma_batt*s*randn;
        case 7  % Extra Drift -- fast-growing bias beyond baseline sensor drift
            faultedVal = trueVal + ExtraDrift_Rate_batt*s*t;
        otherwise
            faultedVal = trueVal;
    end

    % Write the faulted value/valid-flag back into only the targeted channel
    switch target
        case 0
            Battery_Voltage_Final = faultedVal;
            Battery_Voltage_Valid = valid;
        case 1
            Battery_Current_Final = faultedVal;
            Battery_Current_Valid = valid;
        case 2
            Battery_Temperature_Final = faultedVal;
            Battery_Temperature_Valid = valid;
    end
end

end

== matlab function Reformable_AI_2025/PV_Digital_twin/MATLAB Function ==
  data: PV_Measured_Irradiance input; PV_Twin_Current output; PV_Measured_Temperature input; PV_Measured_Voltage input; PV_Twin_Power output; PV_Twin_Rs parameter; PV_Twin_Rsh parameter; PV_Twin_Iph_ref parameter; PV_Twin_I0_ref parameter; PV_Twin_n parameter; PV_Twin_Ns parameter; PV_Twin_Ki parameter; PV_Twin_Eg parameter; PV_Twin_Tref parameter; PV_Twin_Gref parameter; k_B parameter; q parameter
function [PV_Twin_Current, PV_Twin_Power] = ...
    fcn(PV_Measured_Irradiance, PV_Measured_Temperature, PV_Measured_Voltage, ...
        PV_Twin_Rs, PV_Twin_Rsh, PV_Twin_Iph_ref, PV_Twin_I0_ref, ...
PV_Twin_n, PV_Twin_Ns, PV_Twin_Ki, PV_Twin_Eg, PV_Twin_Tref, PV_Twin_Gref, ...
k_B, q)

% TwinAdapt-PHM Stage 8 (Step 1): PV_Digital_Twin
% Independent physics-informed expected-behavior model. Does NOT read
% PV_model's Rs/Rsh/Iph_ref/I0_ref, degradation state, or fault state --
% only observable sensor measurements (irradiance, temperature, voltage)
% and its own independently-named PV_Twin_* parameters.
%
% Re-derives Iph/I0 at the MEASURED operating condition from its own
% reference parameters (same physics as the physical model uses, but
% recalculated independently) -- this is what makes it a genuine Twin
% rather than a lookup of an already-known answer.
%
% Uses PV_Measured_Voltage as the operating point (per Stage 8 Section 11)
% and solves the implicit single-diode equation for current via a fixed
% number of Newton-Raphson iterations -- deterministic, no toolbox
% dependency, safe for a MATLAB Function block.
%
% NOTE ON SYMBOLS PANE: PV_Measured_Irradiance, PV_Measured_Temperature,
% PV_Measured_Voltage must be Scope = Input. Everything after that
% (PV_Twin_Rs ... q) must be Scope = Parameter, resolved from
% PV_Twin_Params.mat.

G = PV_Measured_Irradiance;
Tc_C = PV_Measured_Temperature;
V = PV_Measured_Voltage;

T_K = Tc_C + 273.15;

% --- Re-derive Iph and I0 at the measured operating condition ---
Iph = PV_Twin_Iph_ref * (G/PV_Twin_Gref) * (1 + PV_Twin_Ki*(T_K - PV_Twin_Tref));

I0 = PV_Twin_I0_ref * (T_K/PV_Twin_Tref)^3 * ...
     exp((q*PV_Twin_Eg/(PV_Twin_n*k_B)) * (1/PV_Twin_Tref - 1/T_K));

Vt = PV_Twin_n * PV_Twin_Ns * k_B * T_K / q;

% --- Solve the implicit single-diode equation for current at V ---
% f(I) = Iph - I0*(exp((V+I*Rs)/Vt) - 1) - (V+I*Rs)/Rsh - I = 0
I = Iph;   % initial guess: short-circuit-ish current
for k = 1:8
    expTerm = exp((V + I*PV_Twin_Rs)/Vt);
    f  = Iph - I0*(expTerm - 1) - (V + I*PV_Twin_Rs)/PV_Twin_Rsh - I;
    fp = -I0*(PV_Twin_Rs/Vt)*expTerm - PV_Twin_Rs/PV_Twin_Rsh - 1;
    I = I - f/fp;
end

PV_Twin_Current = I;
PV_Twin_Power   = V * I;

end

== matlab function Reformable_AI_2025/PV_Resdual_Model/MATLAB Function ==
  data: PV_Measured_Current input; PV_Residual_Current output; PV_Twin_Current input; PV_Measured_Power input; PV_Twin_Power input; PV_Residual_Power output
function [PV_Residual_Current, PV_Residual_Power] = ...
    fcn(PV_Measured_Current, PV_Twin_Current, PV_Measured_Power, PV_Twin_Power)

% TwinAdapt-PHM Stage 8 (Step 2): PV_Residual_Model
% Raw residual = measured - twin. No normalization yet (Stage 8 Section 21:
% preserve raw residuals first; normalization, if added later, gets its
% own explicit scale parameters in reformable_AI.m, e.g.
% PV_Residual_Current_Scale / PV_Residual_Power_Scale).
%
% This is not diagnosis -- a nonzero residual here can come from asset
% degradation, an asset fault, a sensor fault, or Twin model mismatch.
% Distinguishing those is later-stage work; this block only computes the
% discrepancy.
%
% NOTE ON SYMBOLS PANE: all 4 arguments are Scope = Input. No parameters.

PV_Residual_Current = PV_Measured_Current - PV_Twin_Current;
PV_Residual_Power   = PV_Measured_Power - PV_Twin_Power;

end

== matlab function Reformable_AI_2025/Battery_Digital_Twin/MATLAB Function ==
  data: Battery_Measured_Current input; Battery_Twin_Voltage output; Battery_Twin_dVp_dt output; Battery_Twin_R0 parameter; Battery_Twin_R1 parameter; Battery_Twin_C1 parameter; Battery_Twin_SOC_bp parameter; Battery_Twin_OCV_tbl parameter; Battery_Twin_SOC_Estimate input; Battery_Twin_Vp input
function [Battery_Twin_Voltage, Battery_Twin_dVp_dt] = ...
    fcn(Battery_Measured_Current, Battery_Twin_R0, Battery_Twin_R1, Battery_Twin_C1, ...
Battery_Twin_SOC_bp, Battery_Twin_OCV_tbl, Battery_Twin_SOC_Estimate, Battery_Twin_Vp) ...

% TwinAdapt-PHM Stage 8 (Step 3): Battery_Digital_Twin -- algebra block
% This is NOT the whole subsystem -- it sits between two Simulink
% Integrator blocks (built-in, not MATLAB code) that hold the Twin's two
% states: SOC estimate and polarization voltage Vp. See the accompanying
% build notes for exactly how to wire it.
%
% Uses OCV source -> R0 -> R1||C1 -> terminal, same topology as the
% physical Battery_Model, but computed independently: reads only
% Battery_Measured_Current (observable) plus its own PV_Twin_* --
% sorry, Battery_Twin_* -- parameters, and its own two integrator states
% fed back in. Never reads True_Battery_Voltage, R0_aged/R1_aged/Q,
% Battery_Health_State, or any hidden fault/degradation signal.
%
% Battery_Twin_SOC_Estimate and Battery_Twin_Vp are NOT inputs from
% outside the subsystem -- they are this same block's own Integrator
% outputs, wired back in. That's what makes them states, not measurements.
% This is not an algebraic loop: each Integrator's OUTPUT at this instant
% is already known before this function runs; only the DERIVATIVE goes
% back out to be integrated forward to the next instant.
%
% NOTE ON SYMBOLS PANE: Battery_Measured_Current, Battery_Twin_SOC_Estimate,
% Battery_Twin_Vp must be Scope = Input. Everything after that
% (Battery_Twin_R0 ... Battery_Twin_OCV_tbl) must be Scope = Parameter,
% resolved from Battery_Twin_Params.mat. Battery_Twin_SOC_bp and
% Battery_Twin_OCV_tbl are vectors -- Parameter scope handles this fine.

OCV = interp1(Battery_Twin_SOC_bp, Battery_Twin_OCV_tbl, Battery_Twin_SOC_Estimate, ...
              'linear', 'extrap');

% Terminal voltage: OCV - drop across R0 - drop across the R1||C1 branch.
% Same sign convention as the physical model: positive current = discharge,
% causing terminal voltage to sag below OCV.
Battery_Twin_Voltage = OCV - Battery_Measured_Current*Battery_Twin_R0 - Battery_Twin_Vp;

% Polarization-voltage state derivative (R1||C1 branch driven by current):
% dVp/dt = I/C1 - Vp/(R1*C1)
Battery_Twin_dVp_dt = Battery_Measured_Current/Battery_Twin_C1 - ...
                      Battery_Twin_Vp/(Battery_Twin_R1*Battery_Twin_C1);

end

== matlab function Reformable_AI_2025/Battery_Residual_Model/MATLAB Function ==
  data: Battery_Measured_Voltage input; Battery_Residual_Voltage output; Battery_Twin_Voltage input
function Battery_Residual_Voltage = ...
    fcn(Battery_Measured_Voltage, Battery_Twin_Voltage)

% TwinAdapt-PHM Stage 8 (Step 4): Battery_Residual_Model
% Raw residual = measured - twin. No normalization yet (same reasoning as
% PV_Residual_Model: Stage 8 Section 21 says preserve raw residuals first).
%
% Only a voltage residual, per Stage 8 Section 20 -- no current residual,
% since Battery_Digital_Twin doesn't produce a defensible independent
% current prediction (current is this Twin's INPUT, not something it
% forecasts). Don't add one just to make PV/Battery symmetrical.
%
% This is not diagnosis -- a nonzero residual here can come from asset
% degradation, an asset fault, a sensor fault, or Twin model mismatch.
% Distinguishing those is later-stage work.
%
% NOTE ON SYMBOLS PANE: both arguments are Scope = Input. No parameters.

Battery_Residual_Voltage = Battery_Measured_Voltage - Battery_Twin_Voltage;

end

== matlab function Reformable_AI_2025/PV_Feature_Engineering/MATLAB Function ==
  data: PV_Residual_Current input; PV_AbsResidual_Current output; PV_Residual_Power input; PV_Measured_Irradiance input; PV_AbsResidual_Power output; PV_Normalized_Current_Residual output; PV_Normalized_Power_Residual output; PV_Valid_Operating_Condition output; Isc_ref parameter; Stage9_Min_Irradiance parameter; Pmax_ref parameter
function [PV_AbsResidual_Current, PV_AbsResidual_Power, ...
          PV_Normalized_Current_Residual, PV_Normalized_Power_Residual, ...
          PV_Valid_Operating_Condition] = ...
    fcn(PV_Residual_Current, PV_Residual_Power, PV_Measured_Irradiance, ...
        Isc_ref, Stage9_Min_Irradiance, Pmax_ref)

% TwinAdapt-PHM Stage 9 (Step 1): PV_Feature_Engineering -- Group A+B
% Instantaneous residual features (normalized) and magnitude features.
% No temporal state here -- purely a function of this instant's inputs.
%
% Normalization denominator is a FIXED nameplate rating (Isc_ref /
% Pmax_ref), never a live signal -- this is what keeps the division
% always safe, regardless of what PV_Twin_Current is doing at low
% irradiance. PV_Valid_Operating_Condition is a SEPARATE interpretive
% flag (not a divide-by-zero guard): it tells later PHM stages "the panel
% is barely generating right now, weigh this residual accordingly" --
% it does NOT silently clip or hide the underlying value.
%
% Deployment-observable: yes. Uses only measured/residual signals plus
% fixed nameplate constants, no hidden ground truth.
%
% NOTE ON SYMBOLS PANE: PV_Residual_Current, PV_Residual_Power,
% PV_Measured_Irradiance must be Scope = Input. Isc_ref, Pmax_ref,
% Stage9_Min_Irradiance must be Scope = Parameter (Isc_ref/Pmax_ref
% already exist in the base workspace from Stage 1 -- reused as-is here
% since they are fixed nameplate constants, not mutable model state).

PV_AbsResidual_Current = abs(PV_Residual_Current);
PV_AbsResidual_Power   = abs(PV_Residual_Power);

PV_Normalized_Current_Residual = PV_Residual_Current / Isc_ref;
PV_Normalized_Power_Residual   = PV_Residual_Power / Pmax_ref;

PV_Valid_Operating_Condition = PV_Measured_Irradiance >= Stage9_Min_Irradiance;

end
